simulink model "modele_decodeur_hamming"  (R2024b)
settings: Solver=FixedStepDiscrete  StartTime=0.0  StopTime=7*Nw*Tc  FixedStep=Tc  RelTol=1e-3
undefined symbols (not defined in the file or in its folder): Tc
settings Model: Creator=youka  LastModifiedBy=youka

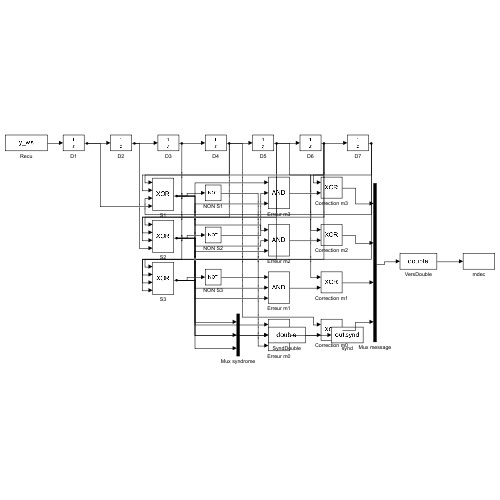
[thumbnail: Simulink's stored preview of the top-level diagram]
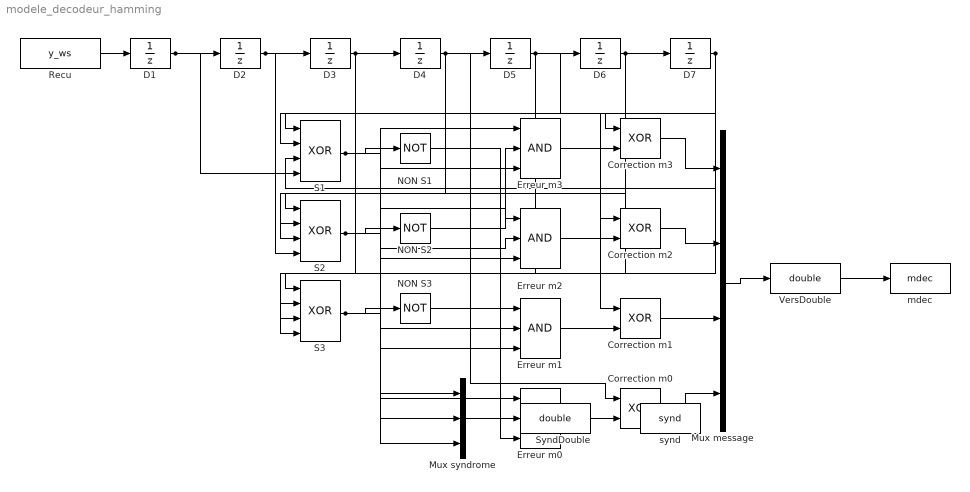
== system modele_decodeur_hamming ==
  Correction m{0..3} (4 alike) : Logic  Operator=XOR  AllPortsSameDT=off  OutDataTypeStr=boolean
  D{1..7} (7 alike) : UnitDelay  SampleTime=Tc  HasFrameUpgradeWarning=on
  Erreur m{0..3} (4 alike) : Logic  Inputs=3  AllPortsSameDT=off  OutDataTypeStr=boolean
  Mux message : Mux
  Mux syndrome : Mux  Inputs=3
  NON S1 : Logic  Operator=NOT  AllPortsSameDT=off  OutDataTypeStr=boolean
  NON S2 : Logic  Operator=NOT  AllPortsSameDT=off  OutDataTypeStr=boolean
  NON S3 : Logic  Operator=NOT  AllPortsSameDT=off  OutDataTypeStr=boolean
  Recu : FromWorkspace  VariableName=y_ws  SampleTime=Tc  Interpolate=off  OutputAfterFinalValue=Setting to zero
  S1 : Logic  Operator=XOR  Inputs=4  AllPortsSameDT=off  OutDataTypeStr=boolean
  S2 : Logic  Operator=XOR  Inputs=4  AllPortsSameDT=off  OutDataTypeStr=boolean
  S3 : Logic  Operator=XOR  Inputs=4  AllPortsSameDT=off  OutDataTypeStr=boolean
  SyndDouble : DataTypeConversion  OutDataTypeStr=double  SaturateOnIntegerOverflow=off  RndMeth=Floor
  VersDouble : DataTypeConversion  OutDataTypeStr=double  SaturateOnIntegerOverflow=off  RndMeth=Floor
  mdec : ToWorkspace  VariableName=mdec  SampleTime=-1
  synd : ToWorkspace  VariableName=synd  SampleTime=-1
  wires:
  Recu/1 -> D1/1
  D1/1 -> D2/1, S1/4
  D2/1 -> D3/1, S2/4
  D3/1 -> D4/1, S3/4
  D4/1 -> D5/1, S1/1, S2/1, Correction m0/1
  D5/1 -> D6/1, S2/2, S3/1, Correction m1/1
  D6/1 -> D7/1, S1/2, S2/3, S3/2, Correction m2/1
  D7/1 -> S1/3, S3/3, Correction m3/1
  S1/1 -> NON S1/1, Erreur m3/1, Erreur m2/1, Erreur m0/1, Mux syndrome/1
  S2/1 -> NON S2/1, Erreur m2/2, Erreur m1/2, Erreur m0/2, Mux syndrome/2
  S3/1 -> NON S3/1, Erreur m3/3, Erreur m2/3, Erreur m1/3, Mux syndrome/3
  NON S2/1 -> Erreur m3/2
  Erreur m3/1 -> Correction m3/2
  Erreur m2/1 -> Correction m2/2
  NON S1/1 -> Erreur m1/1
  Erreur m1/1 -> Correction m1/2
  NON S3/1 -> Erreur m0/3
  Erreur m0/1 -> Correction m0/2
  Correction m3/1 -> Mux message/1
  Correction m2/1 -> Mux message/2
  Correction m1/1 -> Mux message/3
  Correction m0/1 -> Mux message/4
  Mux message/1 -> VersDouble/1
  VersDouble/1 -> mdec/1
  Mux syndrome/1 -> SyndDouble/1
  SyndDouble/1 -> synd/1
